simulink model "sfb_ccc_"  (R2024b)
settings: Solver=FixedStepAuto  StartTime=0.0  StopTime=Ts  FixedStep=Ts  RelTol=1e-3
InitFcn:
  | load('.\data_smk_\fb_c_controller_parameters.mat')
settings Model: Creator=rmrane  LastModifiedBy=vreyesdreke
settings OptimizationCC: DefaultParameterBehavior=Inlined  EnhancedBackFolding=on  PassReuseOutputArgsAs=Individual arguments  ZeroExternalMemoryAtStartup=off  ZeroInternalMemoryAtStartup=off  OptimizeBlockOrder=speed  DifferentSizesBufferReuse=on  OptimizationCustomize=off  EfficientTunableParamExpr=on
settings DebuggingCC: ParameterTunabilityLossMsg=error
settings SFSimCC: MATLABDynamicMemAlloc=off
settings RTWCC: Description=Embedded Coder  SystemTargetFile=ert.tlc  TemplateMakefile=ert_default_tmf
settings CodeAppCC: GenerateComments=off  IgnoreCustomStorageClasses=off  OperatorAnnotations=on  SimulinkDataObjDesc=on  SFDataObjDesc=on  CustomSymbolStrType=$N$R$M  SimulinkBlockComments=off  InternalIdentifier=Classic
settings ERTTargetCC: GenerateSampleERTMain=on  SupportAbsoluteTime=off  SupportNonFinite=off  SupportComplex=off  ERTCustomFileTemplate=example_file_process.tlc  ConvertIfToSwitch=off  SuppressUnreachableDefaultCases=off  EnableSignedLeftShifts=off  EnableSignedRightShifts=off  DynamicArrayContainerType=coder::array

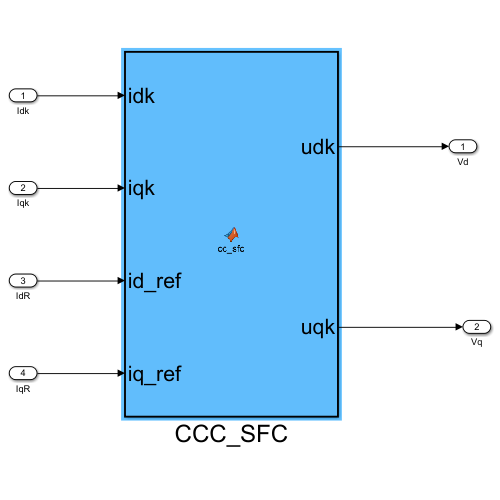
[thumbnail: Simulink's stored preview of the top-level diagram]
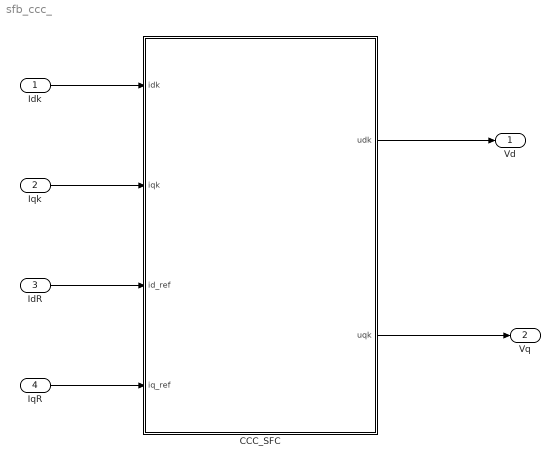
== system sfb_ccc_ ==
  Idk : Inport
  Iqk : Inport  Port=2
  IdR : Inport  Port=3
  IqR : Inport  Port=4
  CCC_SFC : MATLAB Function  TreatAsAtomicUnit=on
  Vd : Outport
  Vq : Outport  Port=2
  wires:
  Idk/1 -> CCC_SFC/1(idk)
  Iqk/1 -> CCC_SFC/2(iqk)
  IdR/1 -> CCC_SFC/3(id_ref)
  IqR/1 -> CCC_SFC/4(iq_ref)
  CCC_SFC/1(udk) -> Vd/1
  CCC_SFC/2(uqk) -> Vq/1

== matlab function sfb_ccc_/CCC_SFC ==
  settings: updateMethod=DISCRETE  sampleTime=Ts
  data: idk input size=1; udk output size=1; uqk output size=1; iqk input size=1; id_ref input size=1; iq_ref input size=1
function [udk,uqk] = cc_sfc(idk, iqk,id_ref,iq_ref)
    % oc_sfc(idk, iqk,id_ref,iq_ref) feedforward controller gain.
    m_ss = coder.load('.\data_smk_\fb_c_controller_parameters.mat','-mat','-regexp','Kfb');
    uk = m_ss.Kfb*([idk, iqk]'-[id_ref,iq_ref]');
    udk = uk(1);
    uqk = uk(2);
end
